simulink model "MainOnLoadDiscrete"  (R2025b)
settings: Solver=VariableStepAuto  StartTime=0.0  StopTime=400  RelTol=1e-3  EnableMultiTasking=on
undefined symbols (not defined in the file or in its folder): DiscIntNeverNeededParam
libraries: slpidlib x4, simulink x2
settings Model: Creator=kkhan  LastModifiedBy=MeisNgan
settings SolverCC: AlgebraicLoopSolver=TrustRegion
settings DataIOCC: ReturnWorkspaceOutputs=off
settings OptimizationCC: LifeSpan=inf
settings DebuggingCC: UnconnectedInputMsg=warning  UnconnectedOutputMsg=warning  UnconnectedLineMsg=warning  SFUnexpectedBacktrackingDiag=warning  SFNoUnconditionalDefaultTransitionDiag=warning  ArithmeticOperatorsInVariantConditions=warning
settings ModelReferenceCC: EnableRefExpFcnMdlSchedulingChecks=on
settings SFSimCC: SimUseLocalCustomCode=off  CustomCodeUndefinedFunction=UseInterfaceOnly
settings RTWCC: RTWUseLocalCustomCode=off  GPUComputeCapability=3.5
settings CodeAppCC: StateflowObjectComments=on
settings GRTTargetCC: TargetLangStandard=C89/C90 (ANSI)
settings ConfigComp: CovMetricSettings=dw  CovSaveCumulativeToWorkspaceVar=on  CovSaveSingleToWorkspaceVar=on  CovExternalEMLEnable=off

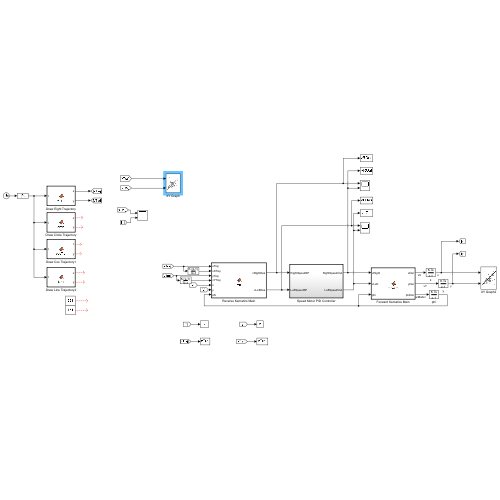
[thumbnail: Simulink's stored preview of the top-level diagram]
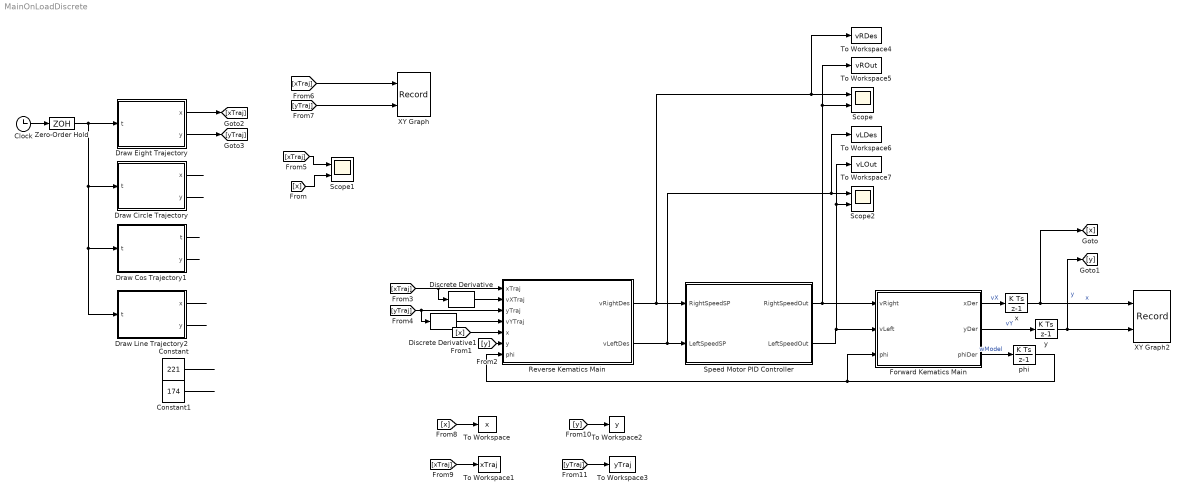
== system MainOnLoadDiscrete ==
  Clock : Clock
  Constant : Constant  Value=221
  Constant1 : Constant  Value=174
  Discrete Derivative : simulink/Discrete/Discrete Derivative  gainval=1  ICPrevScaledInput=0  OutMin=[]  OutMax=[]  OutDataType=fixdt(1, 16)  OutScaling=2^-10  DoSatur=off
  Discrete Derivative1 : simulink/Discrete/Discrete Derivative  gainval=1  ICPrevScaledInput=0  OutMin=[]  OutMax=[]  OutDataType=fixdt(1, 16)  OutScaling=2^-10  DoSatur=off
  Draw Circle Trajectory : MATLAB Function  TreatAsAtomicUnit=on
  Draw Cos Trajectory1 : MATLAB Function  TreatAsAtomicUnit=on
  Draw Eight Trajectory : MATLAB Function  TreatAsAtomicUnit=on
  Draw Line Trajectory2 : MATLAB Function  TreatAsAtomicUnit=on
  Forward Kematics Main : MATLAB Function  TreatAsAtomicUnit=on
  Reverse Kematics Main : MATLAB Function  TreatAsAtomicUnit=on
  Scope : Scope  NumInputPorts=2
      settings: ActiveDisplayYMinimum=-5.74926  ActiveDisplayYMaximum=52.38934  DataLoggingSaveFormat=Array
  Scope1 : Scope  NumInputPorts=2
      settings: ActiveDisplayYMinimum=-375.18537  ActiveDisplayYMaximum=376.23652  DataLoggingVariableName=ScopeData2  DataLoggingSaveFormat=Array
  Scope2 : Scope  NumInputPorts=2
      settings: ActiveDisplayYMinimum=-21.49649  ActiveDisplayYMaximum=37.37372  DataLoggingVariableName=ScopeData3  DataLoggingSaveFormat=Array
  Speed Motor PID Controller : Subsystem  TreatAsAtomicUnit=on
  To Workspace : ToWorkspace  VariableName=x  SaveFormat=Timeseries  SampleTime=-1
      settings: Decimation=2
  To Workspace1 : ToWorkspace  VariableName=xTraj  SaveFormat=Timeseries  SampleTime=-1
      settings: Decimation=2
  To Workspace2 : ToWorkspace  VariableName=y  SaveFormat=Timeseries  SampleTime=-1
      settings: Decimation=2
  To Workspace3 : ToWorkspace  VariableName=yTraj  SaveFormat=Timeseries  SampleTime=-1
      settings: Decimation=2
  To Workspace4 : ToWorkspace  VariableName=vRDes  SaveFormat=Timeseries  SampleTime=-1
      settings: Decimation=2
  To Workspace5 : ToWorkspace  VariableName=vROut  SaveFormat=Timeseries  SampleTime=-1
      settings: Decimation=2
  To Workspace6 : ToWorkspace  VariableName=vLDes  SaveFormat=Timeseries  SampleTime=-1
      settings: Decimation=2
  To Workspace7 : ToWorkspace  VariableName=vLOut  SaveFormat=Timeseries  SampleTime=-1
      settings: Decimation=2
  XY Graph : Record  NumPorts=2.0  FileSettingsInternal="{\"entries\":[{\"content\":{\"excelSettings\":{\"content\":{},\"type\":\"Streamout.ExcelSettings\"},\"parquetSettings\":{\"content\":{},\"type\":\"Streamout.ParquetSettings\"}},\"type\":\"Streamout.FileSettingStorage\",\"uuid\":\"\"}],\"packageUris\":[\"http:\\/\\/schema.mathworks.com\\/mf0\\/streamout_blocks\\/R2020a\"],\"version\":\"1.0\"}"  FrameSettings=[0, 0]  Layout=[1 1]  SignalsInternal="{\"entries\":[{\"content\":{\"signals\":[{\"content\":{\"blockPath\":[],\"dimensions\":[1],\"domain\":\"\",\"lineColor\":\"#a2142f\",\"plots\":[ 1 ],\"port\":1,\"sid\":[\"\"],\"signalID\":1,\"signalName\":\"From6\"},\"type\":\"RecordBlkView.Signal\",\"uuid\":\"\"},{\"content\":{\"blockPath\":[],\"dimensions\":[1],\"domain\":\"\",\"lineColor\":\"#139fff\",\"plots\":[ 1 ],\"port\":2,\"sid\":[\"\"],\"signalID\":2,\"signalName\":\"From7\"},\"type\":\"RecordBlkView.Signal\",\"uuid\":\"\"}]},\"type\":\"RecordBlkView.InputSignals\",\"uuid\":\"\"}],\"packageUris\":[\"http:\\/\\/schema.mathworks.com\\/mf0\\/streamout_blocks\\/R2020a\"],\"version\":\"1.0\"}"  VisualizationBindings="{\"xyplotplugin\":{\"info\":[{\"series\":[{\"bindingParametersList\":[{\"parameter\":\"X-Axis\",\"signalID\":1,\"signalName\":\"From6\"},{\"parameter\":\"Y-Axis\",\"signalID\":2,\"signalName\":\"From7\"}],\"seriesID\":0}],\"subplotID\":1}]}}"  CompatibilityTag=XY  st=0.02
  XY Graph2 : Record  NumPorts=2.0  FileSettingsInternal="{\"entries\":[{\"content\":{\"excelSettings\":{\"content\":{},\"type\":\"Streamout.ExcelSettings\"},\"parquetSettings\":{\"content\":{},\"type\":\"Streamout.ParquetSettings\"}},\"type\":\"Streamout.FileSettingStorage\",\"uuid\":\"\"}],\"packageUris\":[\"http:\\/\\/schema.mathworks.com\\/mf0\\/streamout_blocks\\/R2020a\"],\"version\":\"1.0\"}"  FrameSettings=[0, 0]  Layout=[1 1]  SignalsInternal="{\"entries\":[{\"content\":{\"signals\":[{\"content\":{\"blockPath\":[],\"dimensions\":[1],\"domain\":\"\",\"lineColor\":\"#a2142f\",\"plots\":[ 1 ],\"port\":1,\"sid\":[\"\"],\"signalID\":1,\"signalName\":\"x\"},\"type\":\"RecordBlkView.Signal\",\"uuid\":\"\"},{\"content\":{\"blockPath\":[],\"dimensions\":[1],\"domain\":\"\",\"lineColor\":\"#139fff\",\"plots\":[ 1 ],\"port\":2,\"sid\":[\"\"],\"signalID\":2,\"signalName\":\"y\"},\"type\":\"RecordBlkView.Signal\",\"uuid\":\"\"}]},\"type\":\"RecordBlkView.InputSignals\",\"uuid\":\"\"}],\"packageUris\":[\"http:\\/\\/schema.mathworks.com\\/mf0\\/streamout_blocks\\/R2020a\"],\"version\":\"1.0\"}"  VisualizationBindings="{\"xyplotplugin\":{\"info\":[{\"series\":[{\"bindingParametersList\":[{\"parameter\":\"X-Axis\",\"signalID\":1,\"signalName\":\"x\"},{\"parameter\":\"Y-Axis\",\"signalID\":2,\"signalName\":\"y\"}],\"seriesID\":0}],\"subplotID\":1}]}}"  CompatibilityTag=XY  st=0.02
  Zero-Order Hold : ZeroOrderHold  SampleTime=0.02
  phi : DiscreteIntegrator  SampleTime=0.02  ICPrevOutput=DiscIntNeverNeededParam  ICPrevScaledInput=DiscIntNeverNeededParam
  x : DiscreteIntegrator  SampleTime=0.02  ICPrevOutput=DiscIntNeverNeededParam  ICPrevScaledInput=DiscIntNeverNeededParam
  y : DiscreteIntegrator  SampleTime=0.02  ICPrevOutput=DiscIntNeverNeededParam  ICPrevScaledInput=DiscIntNeverNeededParam
  wires:
  Speed Motor PID Controller/2(LeftSpeedOut) -> To Workspace7/1, Scope2/2, Forward Kematics Main/2(vLeft)
  Forward Kematics Main/1(xDer) -> x/1  "vX"
  Forward Kematics Main/2(yDer) -> y/1  "vY"
  x/1 -> XY Graph2/1, [x]  "x"
  y/1 -> XY Graph2/2, [y]  "y"
  Forward Kematics Main/3(phiDer) -> phi/1  "wModel"
  phi/1 -> Reverse Kematics Main/7(phi), Forward Kematics Main/3(phi)
  Discrete Derivative/1 -> Reverse Kematics Main/2(vXTraj)
  Discrete Derivative1/1 -> Reverse Kematics Main/4(vYTraj)
  [x] -> Scope1/2
  [x] -> Reverse Kematics Main/5(x)
  [y] -> Reverse Kematics Main/6(y)
  [xTraj] -> Discrete Derivative/1, Reverse Kematics Main/1(xTraj)
  [yTraj] -> Discrete Derivative1/1, Reverse Kematics Main/3(yTraj)
  [xTraj] -> Scope1/1
  Draw Circle Trajectory/1(x) -> ?
  Draw Circle Trajectory/2(y) -> ?
  Draw Cos Trajectory1/1(t) -> ?
  Draw Cos Trajectory1/2(y) -> ?
  Draw Line Trajectory2/1(x) -> ?
  Draw Line Trajectory2/2(y) -> ?
  Constant/1 -> ?
  Constant1/1 -> ?
  [x] -> To Workspace/1
  [xTraj] -> To Workspace1/1
  [y] -> To Workspace2/1
  [yTraj] -> To Workspace3/1
  Reverse Kematics Main/1(vRightDes) -> To Workspace4/1, Scope/1, Speed Motor PID Controller/1(RightSpeedSP)
  Speed Motor PID Controller/1(RightSpeedOut) -> Forward Kematics Main/1(vRight), Scope/2, To Workspace5/1
  Reverse Kematics Main/2(vLeftDes) -> To Workspace6/1, Scope2/1, Speed Motor PID Controller/2(LeftSpeedSP)
  [xTraj] -> XY Graph/1
  [yTraj] -> XY Graph/2
  Clock/1 -> Zero-Order Hold/1
  Draw Eight Trajectory/2(y) -> [yTraj]
  Draw Eight Trajectory/1(x) -> [xTraj]
  Zero-Order Hold/1 -> Draw Line Trajectory2/1(t), Draw Cos Trajectory1/1("t "), Draw Circle Trajectory/1(t), Draw Eight Trajectory/1(t)

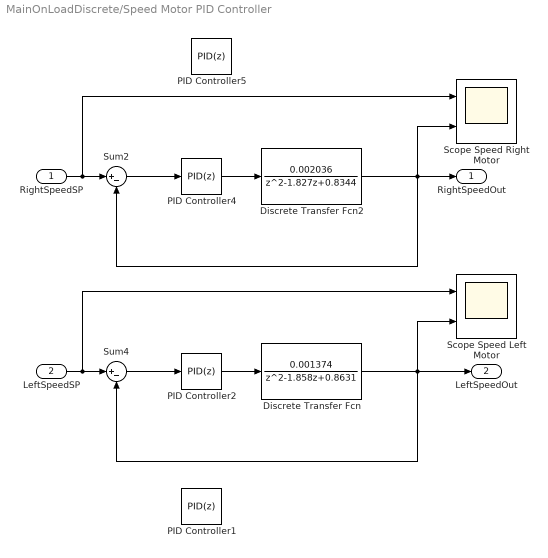
== system MainOnLoadDiscrete/Speed Motor PID Controller ==
  RightSpeedSP : Inport
  LeftSpeedSP : Inport  Port=2
  Discrete Transfer Fcn : DiscreteTransferFcn  Numerator=[0.001374]  Denominator=[1 -1.858 0.8631]  SampleTime=0.02
  Discrete Transfer Fcn2 : DiscreteTransferFcn  Numerator=[0.002036]  Denominator=[1 -1.827 0.8344]  SampleTime=0.02
  PID Controller1 : slpidlib/PID Controller  Controller=PID  Form=Parallel  TimeDomain=Discrete-time  UseExternalTs=off  SampleTime=0.02  IntegratorMethod=Forward Euler  FilterMethod=Forward Euler  ControllerParametersSource=internal  P=17.0258243180127  I=45.6763189239245  UseKiTs=off  D=1.27968580342952  UseExternalDerivativeSource=off  N=83.9177246481862  UseFilter=on  TunerSelectOption=Transfer Function Based (PID Tuner App)  InitialConditionSource=internal  InitialConditionForIntegrator=0  InitialConditionForFilter=0  DifferentiatorICPrevScaledInput=0  ExternalReset=none  TrackingMode=off  Kt=1  LimitOutput=off  SatLimitsSource=internal  UpperSaturationLimit=inf  LowerSaturationLimit=-inf  LinearizeAsGain=on  AntiWindupMode=none  Kb=1  LimitIntegrator=off  UpperIntegratorSaturationLimit=inf  LowerIntegratorSaturationLimit=-inf  POutMin=[]  POutMax=[]  IOutMin=[]  IOutMax=[]  DOutMin=[]  DOutMax=[]  NOutMin=[]  NOutMax=[]  SumOutMin=[]  SumOutMax=[]  SaturationOutMin=[]  SaturationOutMax=[]  PParamMin=[]  PParamMax=[]  IParamMin=[]  IParamMax=[]  DParamMin=[]  DParamMax=[]  NParamMin=[]  NParamMax=[]  KbParamMin=[]  KbParamMax=[]  KtParamMin=[]  KtParamMax=[]  KbOutMin=[]  KbOutMax=[]  KtOutMin=[]  KtOutMax=[]  IntegratorOutMin=[]  IntegratorOutMax=[]  FilterOutMin=[]  FilterOutMax=[]  SumI1OutMin=[]  SumI1OutMax=[]  SumI2OutMin=[]  SumI2OutMax=[]  SumI3OutMin=[]  SumI3OutMax=[]  SumI4OutMin=[]  SumI4OutMax=[]  SumDOutMin=[]  SumDOutMax=[]  DifferentiatorOutMin=[]  DifferentiatorOutMax=[]  FilterDiffOutCoefMin=[]  FilterDiffOutCoefMax=[]  ReciprocalOutMin=[]  ReciprocalOutMax=[]  SumDenOutMin=[]  SumDenOutMax=[]  SumNumOutMin=[]  SumNumOutMax=[]  DivideOutMin=[]  DivideOutMax=[]  UdiffTsProdOutMin=[]  UdiffTsProdOutMax=[]  NTsProdOutMin=[]  NTsProdOutMax=[]  UintegralTsProdOutMin=[]  UintegralTsProdOutMax=[]  UngainTsProdOutMin=[]  UngainTsProdOutMax=[]  ClampingZeroOutDataTypeStr=Inherit: Inherit via back propagation  ClampingZeroOutMin=[]  ClampingZeroOutMax=[]  FilterDenConstantOutDataTypeStr=Inherit: Inherit via back propagation  FilterDenConstantOutMin=[]  FilterDenConstantOutMax=[]  PCopyOutDataTypeStr=Inherit: Inherit via back propagation  PCopyOutMin=[]  PCopyOutMax=[]  NCopyOutDataTypeStr=Inherit: Inherit via back propagation  NCopyOutMin=[]  NCopyOutMax=[]  IntegratorContinuousStateAttributes=''  IntegratorStateMustResolveToSignalObject=off  IntegratorRTWStateStorageClass=Auto  FilterContinuousStateAttributes=''  FilterStateMustResolveToSignalObject=off  FilterRTWStateStorageClass=Auto  ParallelPVariant=InternalParameters  IdealPVariant=Disabled  IVariant=InternalParameters  DVariant=InternalParameters  IntegratorVariant=Discrete  SatVariant=Disabled  AWVariant=Passthrough  PCopyVariant=Disabled  TRVariant=Disabled  FdbkBlocksVariant=Forward  IdealPFdbkVariant=Disabled  SatFdbkVariant=Disabled  DerivativeFilterVariant=ForwardEulerFilter  NVariant=InternalParameters  NCopyVariant=Disabled  FilterICVariant=InternalICsFilter  IntegratorICVariant=InternalICs  ExternalResetVariant=Disabled  TRSumVariant=Passthrough  SumFdbkVariant=Disabled  SumVariant=Sum_PID  TsampFilterVariant=InternalTs  TsampNgainVariant=Passthrough  TsampIntegralVariant=Disabled_SignalSpec  ExternalSaturationOutDataTypeStr=Inherit: Same as second input  DerivativeSourceVariant=ErrorSignal  PreIntVariant=InternalPreInt
  PID Controller2 : slpidlib/PID Controller  Controller=PID  Form=Parallel  TimeDomain=Discrete-time  UseExternalTs=off  SampleTime=0.02  IntegratorMethod=Forward Euler  FilterMethod=Forward Euler  ControllerParametersSource=internal  P=21.0909852919714  I=43.5478218388463  UseKiTs=off  D=2.15960697462874  UseExternalDerivativeSource=off  N=26.7883535297543  UseFilter=on  TunerSelectOption=Transfer Function Based (PID Tuner App)  InitialConditionSource=internal  InitialConditionForIntegrator=0  InitialConditionForFilter=0  DifferentiatorICPrevScaledInput=0  ExternalReset=none  TrackingMode=off  Kt=1  LimitOutput=off  SatLimitsSource=internal  UpperSaturationLimit=inf  LowerSaturationLimit=-inf  LinearizeAsGain=on  AntiWindupMode=none  Kb=1  LimitIntegrator=off  UpperIntegratorSaturationLimit=inf  LowerIntegratorSaturationLimit=-inf  POutMin=[]  POutMax=[]  IOutMin=[]  IOutMax=[]  DOutMin=[]  DOutMax=[]  NOutMin=[]  NOutMax=[]  SumOutMin=[]  SumOutMax=[]  SaturationOutMin=[]  SaturationOutMax=[]  PParamMin=[]  PParamMax=[]  IParamMin=[]  IParamMax=[]  DParamMin=[]  DParamMax=[]  NParamMin=[]  NParamMax=[]  KbParamMin=[]  KbParamMax=[]  KtParamMin=[]  KtParamMax=[]  KbOutMin=[]  KbOutMax=[]  KtOutMin=[]  KtOutMax=[]  IntegratorOutMin=[]  IntegratorOutMax=[]  FilterOutMin=[]  FilterOutMax=[]  SumI1OutMin=[]  SumI1OutMax=[]  SumI2OutMin=[]  SumI2OutMax=[]  SumI3OutMin=[]  SumI3OutMax=[]  SumI4OutMin=[]  SumI4OutMax=[]  SumDOutMin=[]  SumDOutMax=[]  DifferentiatorOutMin=[]  DifferentiatorOutMax=[]  FilterDiffOutCoefMin=[]  FilterDiffOutCoefMax=[]  ReciprocalOutMin=[]  ReciprocalOutMax=[]  SumDenOutMin=[]  SumDenOutMax=[]  SumNumOutMin=[]  SumNumOutMax=[]  DivideOutMin=[]  DivideOutMax=[]  UdiffTsProdOutMin=[]  UdiffTsProdOutMax=[]  NTsProdOutMin=[]  NTsProdOutMax=[]  UintegralTsProdOutMin=[]  UintegralTsProdOutMax=[]  UngainTsProdOutMin=[]  UngainTsProdOutMax=[]  ClampingZeroOutDataTypeStr=Inherit: Inherit via back propagation  ClampingZeroOutMin=[]  ClampingZeroOutMax=[]  FilterDenConstantOutDataTypeStr=Inherit: Inherit via back propagation  FilterDenConstantOutMin=[]  FilterDenConstantOutMax=[]  PCopyOutDataTypeStr=Inherit: Inherit via back propagation  PCopyOutMin=[]  PCopyOutMax=[]  NCopyOutDataTypeStr=Inherit: Inherit via back propagation  NCopyOutMin=[]  NCopyOutMax=[]  IntegratorContinuousStateAttributes=''  IntegratorStateMustResolveToSignalObject=off  IntegratorRTWStateStorageClass=Auto  FilterContinuousStateAttributes=''  FilterStateMustResolveToSignalObject=off  FilterRTWStateStorageClass=Auto  ParallelPVariant=InternalParameters  IdealPVariant=Disabled  IVariant=InternalParameters  DVariant=InternalParameters  IntegratorVariant=Discrete  SatVariant=Disabled  AWVariant=Passthrough  PCopyVariant=Disabled  TRVariant=Disabled  FdbkBlocksVariant=Forward  IdealPFdbkVariant=Disabled  SatFdbkVariant=Disabled  DerivativeFilterVariant=ForwardEulerFilter  NVariant=InternalParameters  NCopyVariant=Disabled  FilterICVariant=InternalICsFilter  IntegratorICVariant=InternalICs  ExternalResetVariant=Disabled  TRSumVariant=Passthrough  SumFdbkVariant=Disabled  SumVariant=Sum_PID  TsampFilterVariant=InternalTs  TsampNgainVariant=Passthrough  TsampIntegralVariant=Disabled_SignalSpec  ExternalSaturationOutDataTypeStr=Inherit: Same as second input  DerivativeSourceVariant=ErrorSignal  PreIntVariant=InternalPreInt
  PID Controller4 : slpidlib/PID Controller  Controller=PID  Form=Parallel  TimeDomain=Discrete-time  UseExternalTs=off  SampleTime=0.02  IntegratorMethod=Forward Euler  FilterMethod=Forward Euler  ControllerParametersSource=internal  P=16.8217157087944  I=42.6084644082369  UseKiTs=off  D=1.35986407955998  UseExternalDerivativeSource=off  N=26.7883535297543  UseFilter=on  TunerSelectOption=Transfer Function Based (PID Tuner App)  InitialConditionSource=internal  InitialConditionForIntegrator=0  InitialConditionForFilter=0  DifferentiatorICPrevScaledInput=0  ExternalReset=none  TrackingMode=off  Kt=1  LimitOutput=off  SatLimitsSource=internal  UpperSaturationLimit=inf  LowerSaturationLimit=-inf  LinearizeAsGain=on  AntiWindupMode=none  Kb=1  LimitIntegrator=off  UpperIntegratorSaturationLimit=inf  LowerIntegratorSaturationLimit=-inf  POutMin=[]  POutMax=[]  IOutMin=[]  IOutMax=[]  DOutMin=[]  DOutMax=[]  NOutMin=[]  NOutMax=[]  SumOutMin=[]  SumOutMax=[]  SaturationOutMin=[]  SaturationOutMax=[]  PParamMin=[]  PParamMax=[]  IParamMin=[]  IParamMax=[]  DParamMin=[]  DParamMax=[]  NParamMin=[]  NParamMax=[]  KbParamMin=[]  KbParamMax=[]  KtParamMin=[]  KtParamMax=[]  KbOutMin=[]  KbOutMax=[]  KtOutMin=[]  KtOutMax=[]  IntegratorOutMin=[]  IntegratorOutMax=[]  FilterOutMin=[]  FilterOutMax=[]  SumI1OutMin=[]  SumI1OutMax=[]  SumI2OutMin=[]  SumI2OutMax=[]  SumI3OutMin=[]  SumI3OutMax=[]  SumI4OutMin=[]  SumI4OutMax=[]  SumDOutMin=[]  SumDOutMax=[]  DifferentiatorOutMin=[]  DifferentiatorOutMax=[]  FilterDiffOutCoefMin=[]  FilterDiffOutCoefMax=[]  ReciprocalOutMin=[]  ReciprocalOutMax=[]  SumDenOutMin=[]  SumDenOutMax=[]  SumNumOutMin=[]  SumNumOutMax=[]  DivideOutMin=[]  DivideOutMax=[]  UdiffTsProdOutMin=[]  UdiffTsProdOutMax=[]  NTsProdOutMin=[]  NTsProdOutMax=[]  UintegralTsProdOutMin=[]  UintegralTsProdOutMax=[]  UngainTsProdOutMin=[]  UngainTsProdOutMax=[]  ClampingZeroOutDataTypeStr=Inherit: Inherit via back propagation  ClampingZeroOutMin=[]  ClampingZeroOutMax=[]  FilterDenConstantOutDataTypeStr=Inherit: Inherit via back propagation  FilterDenConstantOutMin=[]  FilterDenConstantOutMax=[]  PCopyOutDataTypeStr=Inherit: Inherit via back propagation  PCopyOutMin=[]  PCopyOutMax=[]  NCopyOutDataTypeStr=Inherit: Inherit via back propagation  NCopyOutMin=[]  NCopyOutMax=[]  IntegratorContinuousStateAttributes=''  IntegratorStateMustResolveToSignalObject=off  IntegratorRTWStateStorageClass=Auto  FilterContinuousStateAttributes=''  FilterStateMustResolveToSignalObject=off  FilterRTWStateStorageClass=Auto  ParallelPVariant=InternalParameters  IdealPVariant=Disabled  IVariant=InternalParameters  DVariant=InternalParameters  IntegratorVariant=Discrete  SatVariant=Disabled  AWVariant=Passthrough  PCopyVariant=Disabled  TRVariant=Disabled  FdbkBlocksVariant=Forward  IdealPFdbkVariant=Disabled  SatFdbkVariant=Disabled  DerivativeFilterVariant=ForwardEulerFilter  NVariant=InternalParameters  NCopyVariant=Disabled  FilterICVariant=InternalICsFilter  IntegratorICVariant=InternalICs  ExternalResetVariant=Disabled  TRSumVariant=Passthrough  SumFdbkVariant=Disabled  SumVariant=Sum_PID  TsampFilterVariant=InternalTs  TsampNgainVariant=Passthrough  TsampIntegralVariant=Disabled_SignalSpec  ExternalSaturationOutDataTypeStr=Inherit: Same as second input  DerivativeSourceVariant=ErrorSignal  PreIntVariant=InternalPreInt
  PID Controller5 : slpidlib/PID Controller  Controller=PID  Form=Parallel  TimeDomain=Discrete-time  UseExternalTs=off  SampleTime=0.02  IntegratorMethod=Forward Euler  FilterMethod=Forward Euler  ControllerParametersSource=internal  P=12.7137787264422  I=45.1328798006328  UseKiTs=off  D=0.777904407581587  UseExternalDerivativeSource=off  N=83.9177246481862  UseFilter=on  TunerSelectOption=Transfer Function Based (PID Tuner App)  InitialConditionSource=internal  InitialConditionForIntegrator=0  InitialConditionForFilter=0  DifferentiatorICPrevScaledInput=0  ExternalReset=none  TrackingMode=off  Kt=1  LimitOutput=off  SatLimitsSource=internal  UpperSaturationLimit=inf  LowerSaturationLimit=-inf  LinearizeAsGain=on  AntiWindupMode=none  Kb=1  LimitIntegrator=off  UpperIntegratorSaturationLimit=inf  LowerIntegratorSaturationLimit=-inf  POutMin=[]  POutMax=[]  IOutMin=[]  IOutMax=[]  DOutMin=[]  DOutMax=[]  NOutMin=[]  NOutMax=[]  SumOutMin=[]  SumOutMax=[]  SaturationOutMin=[]  SaturationOutMax=[]  PParamMin=[]  PParamMax=[]  IParamMin=[]  IParamMax=[]  DParamMin=[]  DParamMax=[]  NParamMin=[]  NParamMax=[]  KbParamMin=[]  KbParamMax=[]  KtParamMin=[]  KtParamMax=[]  KbOutMin=[]  KbOutMax=[]  KtOutMin=[]  KtOutMax=[]  IntegratorOutMin=[]  IntegratorOutMax=[]  FilterOutMin=[]  FilterOutMax=[]  SumI1OutMin=[]  SumI1OutMax=[]  SumI2OutMin=[]  SumI2OutMax=[]  SumI3OutMin=[]  SumI3OutMax=[]  SumI4OutMin=[]  SumI4OutMax=[]  SumDOutMin=[]  SumDOutMax=[]  DifferentiatorOutMin=[]  DifferentiatorOutMax=[]  FilterDiffOutCoefMin=[]  FilterDiffOutCoefMax=[]  ReciprocalOutMin=[]  ReciprocalOutMax=[]  SumDenOutMin=[]  SumDenOutMax=[]  SumNumOutMin=[]  SumNumOutMax=[]  DivideOutMin=[]  DivideOutMax=[]  UdiffTsProdOutMin=[]  UdiffTsProdOutMax=[]  NTsProdOutMin=[]  NTsProdOutMax=[]  UintegralTsProdOutMin=[]  UintegralTsProdOutMax=[]  UngainTsProdOutMin=[]  UngainTsProdOutMax=[]  ClampingZeroOutDataTypeStr=Inherit: Inherit via back propagation  ClampingZeroOutMin=[]  ClampingZeroOutMax=[]  FilterDenConstantOutDataTypeStr=Inherit: Inherit via back propagation  FilterDenConstantOutMin=[]  FilterDenConstantOutMax=[]  PCopyOutDataTypeStr=Inherit: Inherit via back propagation  PCopyOutMin=[]  PCopyOutMax=[]  NCopyOutDataTypeStr=Inherit: Inherit via back propagation  NCopyOutMin=[]  NCopyOutMax=[]  IntegratorContinuousStateAttributes=''  IntegratorStateMustResolveToSignalObject=off  IntegratorRTWStateStorageClass=Auto  FilterContinuousStateAttributes=''  FilterStateMustResolveToSignalObject=off  FilterRTWStateStorageClass=Auto  ParallelPVariant=InternalParameters  IdealPVariant=Disabled  IVariant=InternalParameters  DVariant=InternalParameters  IntegratorVariant=Discrete  SatVariant=Disabled  AWVariant=Passthrough  PCopyVariant=Disabled  TRVariant=Disabled  FdbkBlocksVariant=Forward  IdealPFdbkVariant=Disabled  SatFdbkVariant=Disabled  DerivativeFilterVariant=ForwardEulerFilter  NVariant=InternalParameters  NCopyVariant=Disabled  FilterICVariant=InternalICsFilter  IntegratorICVariant=InternalICs  ExternalResetVariant=Disabled  TRSumVariant=Passthrough  SumFdbkVariant=Disabled  SumVariant=Sum_PID  TsampFilterVariant=InternalTs  TsampNgainVariant=Passthrough  TsampIntegralVariant=Disabled_SignalSpec  ExternalSaturationOutDataTypeStr=Inherit: Same as second input  DerivativeSourceVariant=ErrorSignal  PreIntVariant=InternalPreInt
  Scope Speed Left Motor : Scope  NumInputPorts=2
      settings: ActiveDisplayYMinimum=-21.49649  ActiveDisplayYMaximum=37.37372
  Scope Speed Right Motor : Scope  NumInputPorts=2
      settings: ActiveDisplayYMinimum=-11.8123  ActiveDisplayYMaximum=106.31072
  Sum2 : Sum  Inputs=|+-
  Sum4 : Sum  Inputs=|+-
  RightSpeedOut : Outport
  LeftSpeedOut : Outport  Port=2
  wires:
  RightSpeedSP/1 -> Scope Speed Right Motor/1, Sum2/1
  Discrete Transfer Fcn2/1 -> Scope Speed Right Motor/2, RightSpeedOut/1, Sum2/2
  Sum2/1 -> PID Controller4/1
  PID Controller4/1 -> Discrete Transfer Fcn2/1
  LeftSpeedSP/1 -> Scope Speed Left Motor/1, Sum4/1
  Discrete Transfer Fcn/1 -> Scope Speed Left Motor/2, LeftSpeedOut/1, Sum4/2
  Sum4/1 -> PID Controller2/1
  PID Controller2/1 -> Discrete Transfer Fcn/1

== matlab function MainOnLoadDiscrete/Draw Cos Trajectory1 ==
  data: t output; y output; t input
function [t,y] = cosTraj(t)
%#codegen
r = 30
w = pi/32;
y = r*cos(w*t);

== matlab function MainOnLoadDiscrete/Forward Kematics Main ==
  data: vRight input; xDer output; vLeft input; yDer output; phiDer output; phi input
function [xDer,yDer,phiDer] = forward(vRight, vLeft, phi)
%#codegen
%Thong so mo hinh
lWheel = 8;
c = 4;
%Input la van toc [cm/s]
vModel = (vRight + vLeft)/2;
%Van toc goc nay la cua mo hinh
wModel = (vRight - vLeft)/(2*lWheel);

vectorMatrix = [cos(phi), -c*sin(phi);
            sin(phi), c*cos(phi);
            0, 1];
velMatrix = [vModel;wModel];

posMatrix = vectorMatrix*velMatrix;

xDer = posMatrix(1);
yDer = posMatrix(2);
phiDer = posMatrix(3);

== matlab function MainOnLoadDiscrete/Draw Circle Trajectory ==
  data: x output; t input; y output
function [x,y] = circle(t)
%#codegen
r = 200;
w = pi/32;
x = r*cos(w*t);
y = r*sin(w*t);

== matlab function MainOnLoadDiscrete/Reverse Kematics Main ==
  data: xTraj input; vXTraj input; yTraj input; vYTraj input; x input; y input; vRightDes output; vLeftDes output; phi input
function [vRightDes,vLeftDes] = fcn(xTraj,vXTraj,yTraj,vYTraj,x,y,phi)
%#codegen
L = 8;
c = 4;
%Input la toa do x, y
%Tu do dao ham se ra van toc dai [cm/s]
stateMatrix = [cos(phi), sin(phi);
               (-1/c)*sin(phi), (1/c)*cos(phi)];
%velMatrix = stateMatrix*[vXTraj + lx*tanh((kx/lx)*(xTraj-x));
%                         vYTraj + ly*tanh((ky/ly)*(yTraj-y))];
velMatrix = stateMatrix*[vXTraj + (xTraj-x);
                         vYTraj + (yTraj-y)];
M = [1, L; 1, -L];
velRLMatrix = M*velMatrix;

vRightDes = velRLMatrix(1);
vLeftDes = velRLMatrix(2);

== matlab function MainOnLoadDiscrete/Draw Eight Trajectory ==
  data: x output; y output; t input
function [x,y] = eight(t)
%#codegen
a = 300;
b = 300;
w = pi/64;
x = a*sin(w*t);
y = (b/2)*sin(2*w*t);

== matlab function MainOnLoadDiscrete/Draw Line Trajectory2 ==
  data: x output; y output; t input
function [x,y] = Line(t)
%#codegen
x = 17 + 22*t;
y = 1 - 50*t;
